simulink model "reduce_emf_before_speedloop"  (R2024b)
settings: Solver=FixedStepAuto  StartTime=0.0  StopTime=25  FixedStep=Tsim  RelTol=1e-4  EnableMultiTasking=on
InitFcn:
  | clc;
  | clear;
  | %% Parameters of the motor
  | Tsim = 1e-6;
  | Tpwm=1e-4;
  | Ts = 1e-4;
  | R = 1.8665;
  | Rs=1.8665;
  | Ls=8.96e-3;
  | Ld = 8.96e-3;
  | Lq = 8.96e-3;
  | L1=(Ld +Lq )/2;
  | L2=(Lq -Ld )/2;
  | flux = 0.21;
  | F=0.00008;
  | J=0.003;
  | Np=4;
  | fpwm = 10e3;
  | Vdc=311;
  | wn=100;
  | %% Controller limiter                                                           % Maximum torque (Nm)
  | I_max = 7.5;                                                    % Maximum current (A)
  | V_max = Vdc/sqrt(3);
  | 
  | 
  | %% 转速环电流环带宽
  | wspd=20;
  | wcur=500;
  | 
  | %% LESO
  | w0=10000;
  | beta1=2*w0-R/Ld;
  | beta2=w0*w0;
  | %% IF启动
  | Iq_if=7;
  | we_if_acc=300;
  | we_if_max=180;
  | we_switch=150;
model workspace (MAT data in the model file):
  new = 0
undefined symbols (not defined in the file or in its folder): DiscIntNeverNeededParam
libraries: spsDCVoltageSourceLib x1, spsGroundLib x1, spsPermanentMagnetSynchronousMachineLib x1, simulink x1, spsUniversalBridgeLib x1, spspowerguiLib x1
(part 1 of 2)
settings Model: SimulationMode=accelerator  Creator=Lenovo  LastModifiedBy=azx
settings SolverCC: AlgebraicLoopSolver=TrustRegion
settings DataIOCC: ReturnWorkspaceOutputs=off
settings OptimizationCC: ReuseModelBlockBuffer=off
settings DebuggingCC: UnconnectedInputMsg=warning  UnconnectedOutputMsg=warning  UnconnectedLineMsg=warning
settings ModelReferenceCC: EnableRefExpFcnMdlSchedulingChecks=on
settings RTWCC: GPUComputeCapability=3.5

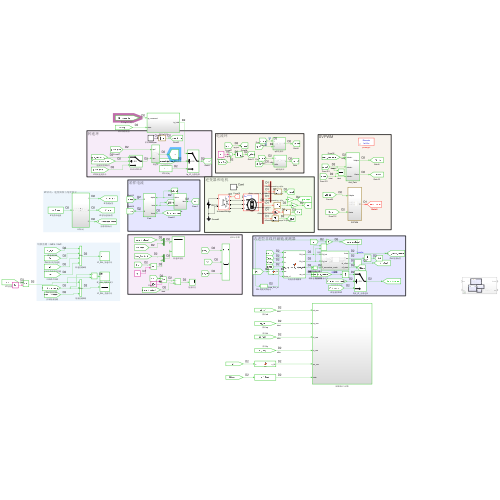
[thumbnail: Simulink's stored preview of the top-level diagram]
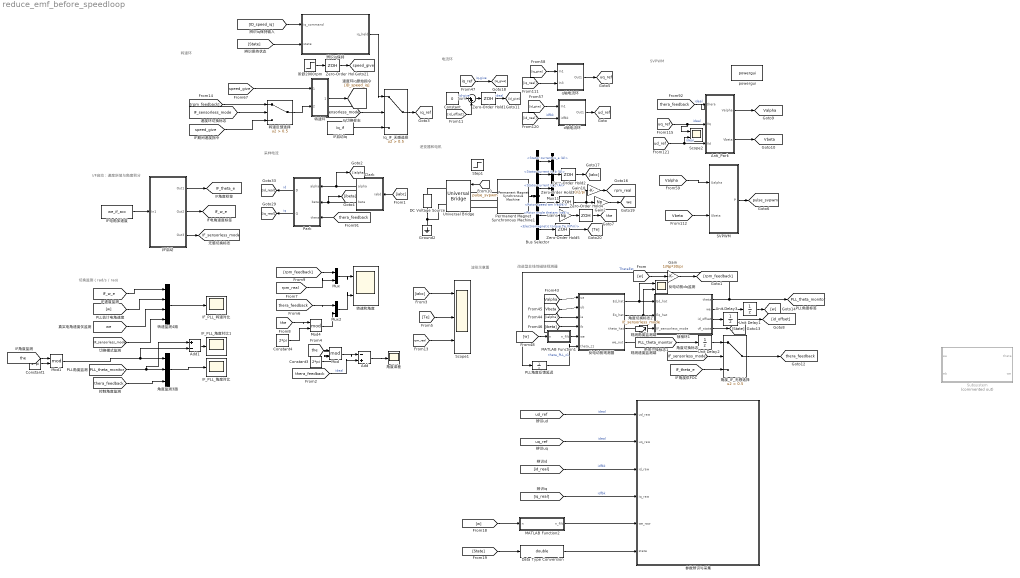
== system reduce_emf_before_speedloop ==
  note: 改进型非线性磁链观测器
  note: 波形示意图
  note: 采样电流
  note: 转速环
  note: SVPWM
  note: 逆变器和电机
  note: 电流环
  note: I/F启动：速度斜坡与角度积分
  note: 切换监测（rad/s / rad）
  Add : Sum  Inputs=-+
  Add1 : Sum  Inputs=+-
  Anti_Park : Subsystem
  Bus Selector : BusSelector  OutputSignals=Stator current is_a (A),Stator current is_b (A),Stator current is_c (A),Rotor speed wm (rad/s),Rotor angle thetam (rad),Electromagnetic torque Te (N*m)
  Clark : Subsystem
  Constant : Constant  Value=0
  Constant1 : Constant  Value=2*pi
  Constant3 : Constant  Value=2*pi
  Constant4 : Constant  Value=2*pi
  DC Voltage Source : spsDCVoltageSourceLib/DC Voltage Source  Amplitude=Vdc  Measurements=None
  Data Type Conversion : DataTypeConversion  OutDataTypeStr=double  SaturateOnIntegerOverflow=off  RndMeth=Floor
  Gain : Gain  Gain=1/Np*30/pi
  Gain10 : Gain  Gain=60/2/pi
  Gain2 : Gain  Gain=Np
  Gain5 : Gain  Gain=Np
  Ground2 : spsGroundLib/Ground  LConnTagsString=a
  I/F启动 : Subsystem
  IF_PLL_角度对比 : Scope
  IF_PLL_角度对比1 : Scope
  IF_PLL_转速对比 : Scope
  IF启动Iq : Constant  Value=Iq_if  SampleTime=Ts
  IF电角加速度 : Constant  Value=we_if_acc  SampleTime=Ts
  Iq_IF_无感选择 : Switch  Criteria=u2 > Threshold  Threshold=0.5
  MATLAB Function1 : MATLAB Function  Description=旁路100Hz低通，使用原有一拍延迟PLL速度，与角度反馈推进严格同拍。  TreatAsAtomicUnit=on
  MATLAB Function2 : MATLAB Function  TreatAsAtomicUnit=on
  Mod : Math  Operator=mod
  Mod1 : Math  Operator=mod
  Mod4 : Math  Operator=mod
  Mux : Mux  Inputs=2
  Mux11 : Mux  Inputs=3
  Mux2 : Mux  Inputs=2
  PLL角度反馈延迟 : UnitDelay  SampleTime=1e-4
  Park : Subsystem
  Permanent Magnet Synchronous Machine1 : spsPermanentMagnetSynchronousMachineLib/Permanent Magnet Synchronous Machine  NbPhases=3  FluxDistribution=Sinusoidal  RotorType=Salient-pole  MechanicalLoad=Torque Tm  PresetModel=No  ShowDetailedParameters=on  MeasurementBus=off  Resistance=R  Inductance=8.5e-3  dqInductances=[Ld,Lq]  La=Ld  MachineConstant=Flux linkage established by magnets (V.s)  Flux=0.21  VoltageCst=152.3591  TorqueCst=1.26  Flat=120  Mechanical=[0.03 2e-2 Np 0]  PolePairs=4  InitialConditions=[0,0, 0,0]  InitialConditions5ph=[0 0 0 0 0 0]  RefAngle=Aligned with phase A axis (original Park)  IterativeDiscreteModel=Trapezoidal non iterative  TsBlock=-1  TsPowergui=0
  SVPWM : Subsystem
  Scope1 : Scope  NumInputPorts=3
  Scope2 : Scope  NumInputPorts=2
  Step1 : Step  Time=0.5  Before=8.5  After=8.5  SampleTime=0
  Subsystem : Subsystem  Commented=on
  Sum : Sum  Inputs=|++
  Unit Delay1 : UnitDelay  SampleTime=-1  HasFrameUpgradeWarning=on
  Unit Delay2 : UnitDelay  SampleTime=-1  HasFrameUpgradeWarning=on
  Unit Delay3 : UnitDelay  SampleTime=-1  HasFrameUpgradeWarning=on
  Universal Bridge : spsUniversalBridgeLib/Universal Bridge  Arms=3  SnubberResistance=1e5  SnubberCapacitance=inf  Device=IGBT / Diodes  Ron=1e-3  Lon=0  ForwardVoltages="[  0  0  ]"  ForwardVoltage=0  GTOparameters=[ 10e-6 , 20e-6 ]  IGBTparameters=[ 1e-6 , 2e-6 ]  Measurements=None  Measurements_2=None  converterType=Rectifier
  Zero-Order Hold{,1..5} (6 alike) : ZeroOrderHold  SampleTime=1e-4
  d轴电流环 : Subsystem
  powergui : spspowerguiLib/powergui  Priority=1  SimulationMode=Discrete  SampleTime=Tsim  frequency=60  Iterations=50  frequencyindice=0  Pbase=100e6  ErrMax=1e-4  UnitsV=kV  UnitsW=MW  buscounter=0  FunctionMessages=off  echomessages=off  EnableUseOfTLC=off  CurrentSourceSwitches=off  DisableSnubberDevices=off  DisableRonSwitches=off  DisableVfSwitches=off  DisplayEquations=off  AutomaticDiscreteSolvers=off  SolverType=Tustin/Backward Euler (TBE)  Interpol=off  ExternalGateDelay=off  methode=off  Ts=100  x0status=blocks  SPID=on  SwTol=0  HookPort=off  NonlinearTolerance=1e-4  nMaxIteration=100  ContinueOnMaxIteration=off  RestoreLinks=warning  ResistiveCurrentMeasurement=off  Frange=[0:2:500]  Ylog=off  Xlog=on  ShowGrid=off  save=off  variable=ZData  structure=0  ZoomFFT=off  StartTime=0.0  cycles=1  DisplayStyle=1  fundamental=60  FreqAxis=off  MaxFrequency=1000  frequencyindicesteady=1  RmsSteady=1  display=off
  q轴电流环 : Subsystem
  参数辨识与采集 : Subsystem
  反电动势dq监测 : Scope  NumInputPorts=2
  反电动势观测器 : MATLAB Function  Description=按文档式12.5-12.7、图12.2实现dq降阶反电动势观测器，Ed/Eq直接送PLL。  TreatAsAtomicUnit=on
  观测角度监测端 : Terminator
  观测速度监测端 : Terminator
  角度_IF_无感选择 : Switch  Criteria=u2 > Threshold  Threshold=0.5
  角度监测3路 : Mux  Inputs=3
  角度误差 : Scope
  转速反馈选择 : Switch  Criteria=u2 > Threshold  Threshold=0.5
  转速和角度 : Scope  NumInputPorts=2
  转速环 : Subsystem
  转速监测4路 : Mux
  辨识iq保持 : Subsystem
  锁相环1 : Subsystem  Description=v2: 每段0.7s，前0.5s稳定、后0.2s采集；2~4与6~8期间保持iq指令，状态9逐点递推。
  阶跃2000rpm : Step  Time=2  Before=500  After=500  SampleTime=0
  tag scope: IF_sensorless_mode=global, IF_theta_e=global, IF_w_e=global, PLL_theta_monitor=global, Valpha=global, Vbeta=global, iq_ref=global, pulse_svpwm=global, rpm_real=global, speed_give=global, the=global, thera_feedback=global, ud_ref=global, uq_ref=global, we=global
  wires:
  [pulse_svpwm] -> Universal Bridge/1
  Clark/2(beta) -> [ibeta], Park/2(beta)
  Clark/1(alpha) -> [ialpha], Park/1(alpha)
  Park/1(D) -> [id_real]  "id"
  Park/2(Q) -> [iq_real]  "iq"
  阶跃2000rpm/1 -> Zero-Order Hold/1
  [thera_feedback] -> Park/3(thera)
  [thera_feedback] -> Anti_Park/1(thera)  "ideal"
  [ud_ref] -> Scope2/2, Anti_Park/3(Vd)  "ideal"
  [uq_ref] -> Scope2/1, Anti_Park/2(Vq)  "ideal"
  [iabc] -> Clark/1(iabd)
  Zero-Order Hold/1 -> [speed_give]
  Zero-Order Hold1/1 -> [id_give]  "ideal"
  Bus Selector/1 -> Mux11/1  "<Stator current is_a (A)>"
  Bus Selector/3 -> Mux11/3  "<Stator current is_c (A)>"
  Zero-Order Hold3/1 -> Gain2/1, Gain10/1
  Zero-Order Hold5/1 -> [Te]
  Gain2/1 -> [we]
  Mux11/1 -> Zero-Order Hold2/1
  Bus Selector/2 -> Mux11/2  "<Stator current is_b (A)>"
  Bus Selector/5 -> Gain5/1  "<Rotor angle thetam (rad)>"
  Bus Selector/4 -> Zero-Order Hold3/1  "<Rotor speed wm (rad/s)>"
  Bus Selector/6 -> Zero-Order Hold5/1  "<Electromagnetic torque Te (N*m)>"
  Zero-Order Hold2/1 -> [iabc]
  Gain10/1 -> [rpm_real]
  Permanent Magnet Synchronous Machine1/1 -> Bus Selector/1
  Zero-Order Hold4/1 -> [the]
  Gain5/1 -> Zero-Order Hold4/1
  [rpm_feedback] -> Mux/1
  [rpm_real] -> Mux/2
  [thera_feedback] -> Mux2/1
  Mux2/1 -> 转速和角度/2
  Mux/1 -> 转速和角度/1
  [the] -> Mod/1
  Constant3/1 -> Mod/2
  Mod/1 -> Add/1
  Add/1 -> 角度误差/1
  Anti_Park/1(Valpha) -> [Valpha]
  Anti_Park/2(Vbeta) -> [Vbeta]
  [thera_feedback] -> Add/2  "ideal"
  [the] -> Mod4/1
  Constant4/1 -> Mod4/2
  Mod4/1 -> Mux2/2
  [speed_give] -> 转速环/1(rpm*)
  [iq_give] -> q轴电流环/1(In1)
  [iq_real] -> q轴电流环/2(In3)
  q轴电流环/1(Out1) -> [uq_ref]
  [id_give] -> d轴电流环/1(In1)
  [id_real] -> d轴电流环/2(idfbk)  "idfbk"
  d轴电流环/1(Out1) -> [ud_ref]
  SVPWM/1(P) -> [pulse_svpwm]
  [rpm_real] -> Scope1/3
  [Te] -> Scope1/2
  [iabc] -> Scope1/1
  Gain/1 -> [rpm_feedback]
  [Valpha] -> 反电动势观测器/1(ua)
  反电动势观测器/2(Eq_hat) -> 锁相环1/2(Eq_hat), 反电动势dq监测/2
  [Vbeta] -> 反电动势观测器/2(ub)
  [ialpha] -> 反电动势观测器/3(ia)
  [ibeta] -> 反电动势观测器/4(ib)
  反电动势观测器/1(Ed_hat) -> 锁相环1/1(Ed_hat), 反电动势dq监测/1
  Unit Delay1/1 -> [w]
  角度_IF_无感选择/1 -> [thera_feedback]
  [Valpha] -> SVPWM/1(Ualpha)
  [Vbeta] -> SVPWM/2(Ubeta)
  锁相环1/2(we) -> Unit Delay1/1
  [w] -> MATLAB Function1/1(n)
  [w] -> Gain/1
  [IF_sensorless_mode] -> Iq_IF_无感选择/2
  IF启动Iq/1 -> Iq_IF_无感选择/3
  Iq_IF_无感选择/1 -> [iq_ref]
  [rpm_feedback] -> 转速反馈选择/1
  [IF_sensorless_mode] -> 转速反馈选择/2
  [speed_give] -> 转速反馈选择/3
  转速反馈选择/1 -> 转速环/2(rpm)
  锁相环1/1(theta) -> [PLL_theta_monitor], PLL角度反馈延迟/1  "ThetaEst"
  [IF_sensorless_mode] -> 角度_IF_无感选择/2
  [IF_theta_e] -> 角度_IF_无感选择/3
  [IF_w_e] -> 转速监测4路/1
  [w] -> 转速监测4路/2
  [we] -> 转速监测4路/3
  [IF_sensorless_mode] -> 转速监测4路/4
  转速监测4路/1 -> IF_PLL_转速对比/1
  [PLL_theta_monitor] -> Add1/1, 角度监测3路/2
  [thera_feedback] -> 角度监测3路/3
  角度监测3路/1 -> IF_PLL_角度对比/1
  [PLL_theta_monitor] -> Unit Delay2/1
  IF电角加速度/1 -> I/F启动/1(In1)
  I/F启动/1(Out1) -> [IF_theta_e]
  I/F启动/2(Out2) -> [IF_w_e]
  I/F启动/3(Out3) -> [IF_sensorless_mode]
  [IF_sensorless_mode] -> 锁相环1/3(IF_sensorless_mode)
  锁相环1/3(id_offset) -> Unit Delay3/1
  Sum/1 -> Zero-Order Hold1/1
  Constant/1 -> Sum/1  "id-give"
  [id_offset] -> Sum/2
  Unit Delay3/1 -> [id_offset]
  [w] -> MATLAB Function2/1(n)
  锁相环1/4(vfl_state) -> [State]
  [State] -> Data Type Conversion/1
  Add1/1 -> IF_PLL_角度对比1/1
  [the] -> Mod1/1
  Constant1/1 -> Mod1/2
  Mod1/1 -> Add1/2, 角度监测3路/1
  MATLAB Function1/1(n_filt) -> 反电动势观测器/5("we ")
  Unit Delay2/1 -> 角度_IF_无感选择/1
  PLL角度反馈延迟/1 -> 反电动势观测器/6(theta_z1)  "theta_PLL_z1"
  反电动势观测器/3(theta_hat) -> 观测角度监测端/1
  反电动势观测器/4(we_out) -> 观测速度监测端/1
  [ud_ref] -> 参数辨识与采集/1(ud_raw)  "ideal"
  [uq_ref] -> 参数辨识与采集/2(uq_raw)  "ideal"
  [id_real] -> 参数辨识与采集/3(id_raw)  "idfbk"
  [iq_real] -> 参数辨识与采集/4(iq_raw)  "idfbk"
  MATLAB Function2/1(n_filt) -> 参数辨识与采集/5(we_raw)
  Data Type Conversion/1 -> 参数辨识与采集/6(state)
  [State] -> 辨识iq保持/2(state)
  辨识iq保持/1(iq_held) -> Iq_IF_无感选择/1
  [iq_ref] -> [iq_give]  "iq-give"
  转速环/1(Out1) -> [ID_speed_iq]
  [ID_speed_iq] -> 辨识iq保持/1(iq_command)
  connections:
  DC Voltage Source/RConn1 -- Universal Bridge/RConn1
  Permanent Magnet Synchronous Machine1/LConn1 -- Universal Bridge/LConn1
  Permanent Magnet Synchronous Machine1/LConn2 -- Universal Bridge/LConn2
  Permanent Magnet Synchronous Machine1/LConn3 -- Universal Bridge/LConn3
  Universal Bridge/RConn2 -- DC Voltage Source/LConn1 -- Ground2/LConn1

== system reduce_emf_before_speedloop/Anti_Park ==
  thera : Inport
  Vq : Inport  Port=2
  Vd : Inport  Port=3
  Fcn : Fcn  Expr=cos(u[1])*u[2]-sin(u[1])*u[3]
  Fcn1 : Fcn  Expr=sin(u[1])*u[2]+cos(u[1])*u[3]
  Mux1 : Mux  Inputs=3
  Valpha : Outport
  Vbeta : Outport  Port=2
  wires:
  thera/1 -> Mux1/1
  Mux1/1 -> Fcn1/1, Fcn/1
  Vq/1 -> Mux1/3
  Fcn1/1 -> Vbeta/1
  Vd/1 -> Mux1/2
  Fcn/1 -> Valpha/1

== system reduce_emf_before_speedloop/Clark ==
  iabd : Inport
  Fcn : Fcn  Expr=(u(1)-0.5*(u(2)+u(3)))*2/3
  Fcn1 : Fcn  Expr=sqrt(3)/2*(u(2)-u(3))*2/3
  alpha : Outport
  beta : Outport  Port=2
  tag scope: Ialpha_real=global, Ibeta_real=global
  wires:
  iabd/1 -> Fcn1/1, Fcn/1
  Fcn/1 -> [Ialpha_real], alpha/1
  Fcn1/1 -> [Ibeta_real], beta/1

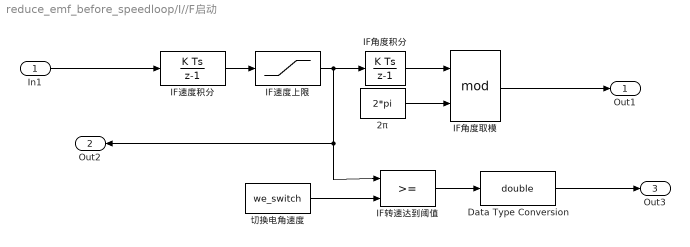
== system reduce_emf_before_speedloop/I//F启动 ==
  In1 : Inport
  2π : Constant  Value=2*pi  SampleTime=Ts
  Data Type Conversion : DataTypeConversion  OutDataTypeStr=double  SaturateOnIntegerOverflow=off  RndMeth=Floor
  IF角度取模 : Math  Operator=mod
  IF角度积分 : DiscreteIntegrator  SampleTime=Ts  ICPrevOutput=DiscIntNeverNeededParam  ICPrevScaledInput=DiscIntNeverNeededParam
  IF转速达到阈值 : RelationalOperator
  IF速度上限 : Saturate  UpperLimit=we_if_max  LowerLimit=0
  IF速度积分 : DiscreteIntegrator  SampleTime=Ts  ICPrevOutput=DiscIntNeverNeededParam  ICPrevScaledInput=DiscIntNeverNeededParam
  切换电角速度 : Constant  Value=we_switch  SampleTime=Ts
  Out1 : Outport
  Out2 : Outport  Port=2
  Out3 : Outport  Port=3
  wires:
  切换电角速度/1 -> IF转速达到阈值/2
  IF速度积分/1 -> IF速度上限/1
  2π/1 -> IF角度取模/2
  IF速度上限/1 -> Out2/1, IF转速达到阈值/1, IF角度积分/1
  IF角度积分/1 -> IF角度取模/1
  IF转速达到阈值/1 -> Data Type Conversion/1
  In1/1 -> IF速度积分/1
  Data Type Conversion/1 -> Out3/1
  IF角度取模/1 -> Out1/1

== system reduce_emf_before_speedloop/Park ==
  alpha : Inport
  beta : Inport  Port=2
  thera : Inport  Port=3
  Fcn : Fcn  Expr=u(1)*cos(u(3))+u(2)*sin(u(3))
  Fcn1 : Fcn  Expr=-u(1)*sin(u(3))+u(2)*cos(u(3))
  Mux1 : Mux  Inputs=3
  D : Outport
  Q : Outport  Port=2
  wires:
  beta/1 -> Mux1/2
  Mux1/1 -> Fcn1/1, Fcn/1
  thera/1 -> Mux1/3
  Fcn/1 -> D/1
  Fcn1/1 -> Q/1
  alpha/1 -> Mux1/1

== system reduce_emf_before_speedloop/SVPWM ==
  Ualpha : Inport
  Ubeta : Inport  Port=2
  Rate Transition : RateTransition  Deterministic=off
  Rate Transition12 : RateTransition  Deterministic=off
  SVPWM : Subsystem
  P : Outport
  wires:
  Ualpha/1 -> Rate Transition/1
  Ubeta/1 -> Rate Transition12/1
  Rate Transition/1 -> SVPWM/1(alpha)
  Rate Transition12/1 -> SVPWM/2(beta)
  SVPWM/1(Pulse) -> P/1

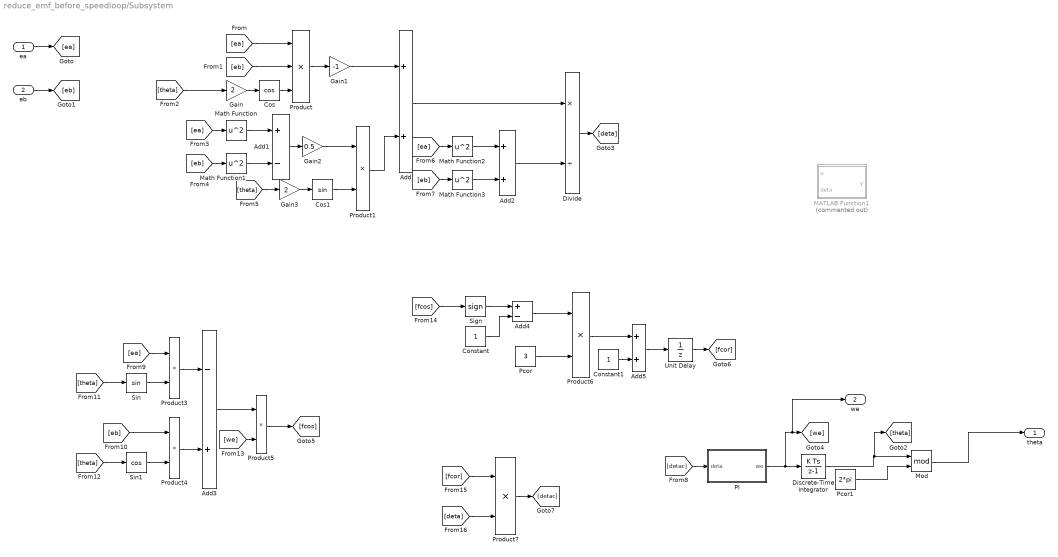
== system reduce_emf_before_speedloop/Subsystem ==
  ea : Inport
  eb : Inport  Port=2
  Add : Sum
  Add1 : Sum  Inputs=+-
  Add2 : Sum
  Add3 : Sum  Inputs=-+
  Add4 : Sum  Inputs=+-
  Add5 : Sum
  Constant : Constant
  Constant1 : Constant
  Cos : Trigonometry  Operator=cos
  Cos1 : Trigonometry
  Discrete-Time Integrator : DiscreteIntegrator  SampleTime=-1  ICPrevOutput=DiscIntNeverNeededParam  ICPrevScaledInput=DiscIntNeverNeededParam
  Divide : Product  Inputs=*/
  Gain : Gain  Gain=2
  Gain1 : Gain  Gain=-1
  Gain2 : Gain  Gain=0.5
  Gain3 : Gain  Gain=2
  MATLAB Function1 : MATLAB Function  Commented=on  TreatAsAtomicUnit=on
  Math Function{,1..3} (4 alike) : Math  Operator=square
  Mod : Math  Operator=mod
  PI : Subsystem
  Pcor : Constant  Value=3
  Pcor1 : Constant  Value=2*pi
  Product : Product  Inputs=3
  Product{1,3..7} (6 alike) : Product
  Sign : Signum
  Sin : Trigonometry
  Sin1 : Trigonometry  Operator=cos
  Unit Delay : UnitDelay  SampleTime=-1  HasFrameUpgradeWarning=on
  theta : Outport
  we : Outport  Port=2
  wires:
  ea/1 -> [ea]
  eb/1 -> [eb]
  [ea] -> Product/1
  [eb] -> Product/2
  Cos/1 -> Product/3
  Gain/1 -> Cos/1
  [theta] -> Gain/1
  Product/1 -> Gain1/1
  Gain1/1 -> Add/1
  [ea] -> Math Function/1
  [eb] -> Math Function1/1
  Math Function/1 -> Add1/1
  Math Function1/1 -> Add1/2
  Add1/1 -> Gain2/1
  Gain2/1 -> Product1/1
  Product1/1 -> Add/2
  Cos1/1 -> Product1/2
  Gain3/1 -> Cos1/1
  [theta] -> Gain3/1
  Add/1 -> Divide/1
  Math Function3/1 -> Add2/2
  [ea] -> Math Function2/1
  [eb] -> Math Function3/1
  Math Function2/1 -> Add2/1
  [ea] -> Product3/1
  Sin/1 -> Product3/2
  [theta] -> Sin/1
  [eb] -> Product4/1
  [theta] -> Sin1/1
  Sin1/1 -> Product4/2
  Product3/1 -> Add3/1
  Product4/1 -> Add3/2
  Add3/1 -> Product5/1
  [we] -> Product5/2
  Product5/1 -> [fcos]
  [fcos] -> Sign/1
  Sign/1 -> Add4/1
  Constant/1 -> Add4/2
  Add4/1 -> Product6/1
  Pcor/1 -> Product6/2
  Product6/1 -> Add5/1
  Constant1/1 -> Add5/2
  Add5/1 -> Unit Delay/1
  [fcor] -> Product7/1
  [deta] -> Product7/2
  Product7/1 -> [detac]
  PI/1(we) -> Discrete-Time Integrator/1, we/1, [we]
  Discrete-Time Integrator/1 -> [theta], Mod/1
  Unit Delay/1 -> [fcor]
  Pcor1/1 -> Mod/2
  [detac] -> PI/1(deta)
  Add2/1 -> Divide/2
  Divide/1 -> [deta]
  Mod/1 -> theta/1

== system reduce_emf_before_speedloop/d轴电流环 ==
  In1 : Inport
  idfbk : Inport  Port=2
  30id : Subsystem  DialogController=POWERSYS.PowerSysDialog  mask(Discrete PI Controller){Kp=2*pi*wcur*Ld, Ki=2*pi*wcur*R, Par_Limits=[V_max -V_max], Init=0, Ts=Ts}
      mask prompts: Kp "Proportional gain (Kp):"; Ki "Integral gain (Ki):"; Par_Limits "Output limits: [ Upper   Lower ]"; Init "Output initial value:"; Ts "Sample time:"
      mask help: This block implements a discrete PI controller.
      mask init:
      | UpperLimit=Par_Limits(1);
      | LowerLimit=Par_Limits(2);
      | power_initmask();
      mask Help: This block is part of a subset of blocks in the Extras library that does not have documentation associated with it, other than the block mask description.
      mask Display: disp('PI');
  Sum1 : Sum  Inputs=|+-
  Sum7 : Sum  Inputs=|+-
  Out1 : Outport
  wires:
  30id/1(Out) -> Sum7/1  "ideal"
  Sum1/1 -> 30id/1(Error)
  Sum7/1 -> Out1/1
  idfbk/1 -> Sum1/2
  In1/1 -> Sum1/1

== system reduce_emf_before_speedloop/q轴电流环 ==
  In1 : Inport
  In3 : Inport  Port=2
  30iq : Subsystem  DialogController=POWERSYS.PowerSysDialog  mask(Discrete PI Controller){Kp=2*pi*wcur*Lq, Ki=2*pi*wcur*R, Par_Limits=[V_max -V_max], Init=0, Ts=Ts}
      mask prompts: Kp "Proportional gain (Kp):"; Ki "Integral gain (Ki):"; Par_Limits "Output limits: [ Upper   Lower ]"; Init "Output initial value:"; Ts "Sample time:"
      mask help: This block implements a discrete PI controller.
      mask init:
      | UpperLimit=Par_Limits(1);
      | LowerLimit=Par_Limits(2);
      | power_initmask();
      mask Help: This block is part of a subset of blocks in the Extras library that does not have documentation associated with it, other than the block mask description.
      mask Display: disp('PI');
  Sum2 : Sum  Inputs=|+-
  Sum6 : Sum  Inputs=|++
  Out1 : Outport
  wires:
  In3/1 -> Sum2/2
  30iq/1(Out) -> Sum6/1  "ideal"
  Sum2/1 -> 30iq/1(Error)
  In1/1 -> Sum2/1
  Sum6/1 -> Out1/1

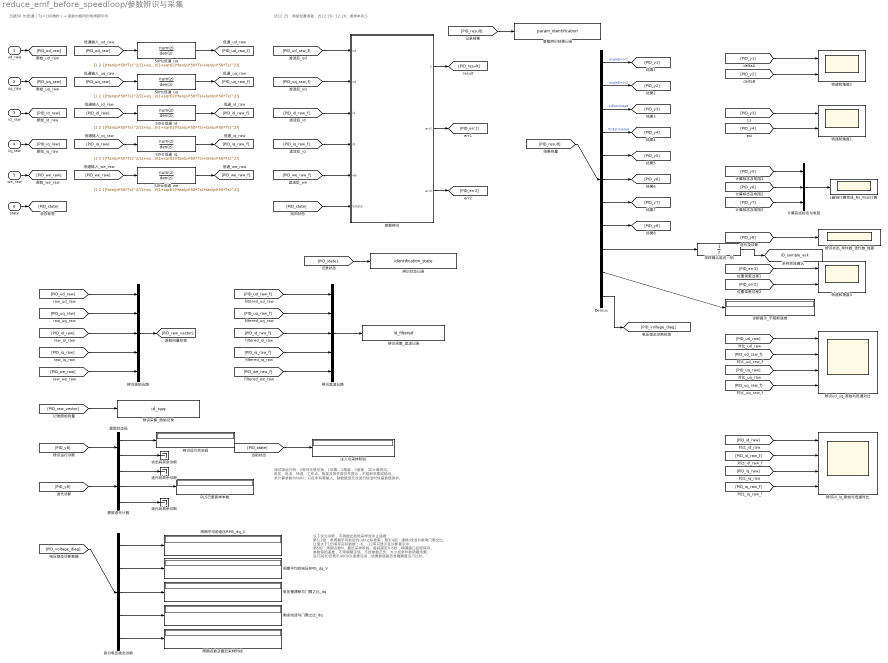
== system reduce_emf_before_speedloop/参数辨识与采集 ==
  note: 五路50 Hz低通（Ts=100微秒）→ 函数内相同的电周期平均
  note: 式12.25：两组位置误差；式12.26～12.28：逐样本RLS
  note: 调试版运行码：0等待无感切换，1采集，2角度，3递推，30计算完成。
      | 电压、电流、转速、工作点、角度及条件数仅作提示，不阻断采集或输出。
      | 未计算参数为NaN；只在非有限输入、缺数据或无法进行除法时保留数值保护。
  note: 以下仅为诊断，不再据此拒绝采样或中止递推：
      | 第1/2组：电周期平均前后的ud/uq标准差；第3/4组：漂移/纹波与参考门限之比。
      | 比值大于1仍保存实际数据；-6、-12等只显示在诊断提示中。
      | 第5组：周期点数N、最近采样阶段。每段固定0.6秒，填满窗口后即保存。
      | 参数每拍递推，不预填额定值，不按参数正负、大小或条件数隐藏结果。
      | 运行码30仅表示4000次递推完成，结果数值是否准确需要另行比对。
  ud_raw : Inport
  uq_raw : Inport  Port=2
  id_raw : Inport  Port=3
  iq_raw : Inport  Port=4
  we_raw : Inport  Port=5
  state : Inport  Port=6
  50Hz低通_id : DiscreteTransferFcn  Description=输入已是Ts=100us；同速率二阶Butterworth低通，不作升采样，不声称恢复上游已混叠信息。  Numerator=[1 2 1]*tan(pi*50*Ts)^2/(1+sqrt(2)*tan(pi*50*Ts)+tan(pi*50*Ts)^2)  Denominator=[1 2*(tan(pi*50*Ts)^2-1)/(1+sqrt(2)*tan(pi*50*Ts)+tan(pi*50*Ts)^2) (1-sqrt(2)*tan(pi*50*Ts)+tan(pi*50*Ts)^2)/(1+sqrt(2)*tan(pi*50*Ts)+tan(pi*50*Ts)^2)]  SampleTime=Ts
  50Hz低通_iq : DiscreteTransferFcn  Description=输入已是Ts=100us；同速率二阶Butterworth低通，不作升采样，不声称恢复上游已混叠信息。  Numerator=[1 2 1]*tan(pi*50*Ts)^2/(1+sqrt(2)*tan(pi*50*Ts)+tan(pi*50*Ts)^2)  Denominator=[1 2*(tan(pi*50*Ts)^2-1)/(1+sqrt(2)*tan(pi*50*Ts)+tan(pi*50*Ts)^2) (1-sqrt(2)*tan(pi*50*Ts)+tan(pi*50*Ts)^2)/(1+sqrt(2)*tan(pi*50*Ts)+tan(pi*50*Ts)^2)]  SampleTime=Ts
  50Hz低通_ud : DiscreteTransferFcn  Description=输入已是Ts=100us；同速率二阶Butterworth低通，不作升采样，不声称恢复上游已混叠信息。  Numerator=[1 2 1]*tan(pi*50*Ts)^2/(1+sqrt(2)*tan(pi*50*Ts)+tan(pi*50*Ts)^2)  Denominator=[1 2*(tan(pi*50*Ts)^2-1)/(1+sqrt(2)*tan(pi*50*Ts)+tan(pi*50*Ts)^2) (1-sqrt(2)*tan(pi*50*Ts)+tan(pi*50*Ts)^2)/(1+sqrt(2)*tan(pi*50*Ts)+tan(pi*50*Ts)^2)]  SampleTime=Ts
  50Hz低通_uq : DiscreteTransferFcn  Description=输入已是Ts=100us；同速率二阶Butterworth低通，不作升采样，不声称恢复上游已混叠信息。  Numerator=[1 2 1]*tan(pi*50*Ts)^2/(1+sqrt(2)*tan(pi*50*Ts)+tan(pi*50*Ts)^2)  Denominator=[1 2*(tan(pi*50*Ts)^2-1)/(1+sqrt(2)*tan(pi*50*Ts)+tan(pi*50*Ts)^2) (1-sqrt(2)*tan(pi*50*Ts)+tan(pi*50*Ts)^2)/(1+sqrt(2)*tan(pi*50*Ts)+tan(pi*50*Ts)^2)]  SampleTime=Ts
  50Hz低通_we : DiscreteTransferFcn  Description=输入已是Ts=100us；同速率二阶Butterworth低通，不作升采样，不声称恢复上游已混叠信息。  Numerator=[1 2 1]*tan(pi*50*Ts)^2/(1+sqrt(2)*tan(pi*50*Ts)+tan(pi*50*Ts)^2)  Denominator=[1 2*(tan(pi*50*Ts)^2-1)/(1+sqrt(2)*tan(pi*50*Ts)+tan(pi*50*Ts)^2) (1-sqrt(2)*tan(pi*50*Ts)+tan(pi*50*Ts)^2)/(1+sqrt(2)*tan(pi*50*Ts)+tan(pi*50*Ts)^2)]  SampleTime=Ts
  Demux : Demux  Outputs=[1 1 1 1 1 1 1 8 1 1 10]
  L磁链计算完成_Rs_Rs已计算 : Scope
  RLS已更新样本数 : Display
  剩余纹波与门限之比_dq : Display
  参数辨识 : MATLAB Function  Description=v7调试版：填满窗口即保存，质量诊断不拒绝数据；按真实存储数据执行4000次递推。运行码30表示递推完成，计算标志不表示通过精度或物理验收。  TreatAsAtomicUnit=on
  参数辨识结果记录 : ToWorkspace  VariableName=param_identification  SaveFormat=Structure With Time  SampleTime=Ts
  周期平均前电压RMS_dq_V : Display
  周期平均后电压RMS_dq_V : Display
  周期点数及最近采样阶段 : Display
  拆分电压稳态诊断 : Demux  Outputs=[2 2 2 2 2]
  提取状态码 : Demux  Outputs=[1 7]
  提取迭代计数 : Demux  Outputs=[4 1 3]
  注入与采样阶段 : Display
  状态码其余诊断 : Terminator
  电压慢漂移与门限之比_dq : Display
  计算完成标志与电阻 : Mux  Inputs=3
  诊断提示_不阻断递推 : Display
  转速和角度1 : Scope  NumInputPorts=2
  转速和角度2 : Scope  NumInputPorts=2
  转速和角度4 : Scope  NumInputPorts=2
  辨识id_iq_原始与低通对比 : Scope
  辨识ud_uq_原始与低通对比 : Scope
  辨识原始五路 : Mux  Inputs=5
  辨识滤波五路 : Mux  Inputs=5
  辨识状态_条件数_迭代数_残差 : Scope
  辨识状态记录 : ToWorkspace  VariableName=identification_state  SaveFormat=Structure With Time  SampleTime=Ts
  辨识运行状态码 : Display
  辨识采集_原始记录 : ToWorkspace  VariableName=id_raw  SaveFormat=Structure With Time  SampleTime=Ts
  辨识采集_滤波记录 : ToWorkspace  VariableName=id_filtered  SaveFormat=Structure With Time  SampleTime=Ts
  迭代前其余诊断 : Terminator
  迭代后其余诊断 : Terminator
  采样确认延迟一拍 : UnitDelay  SampleTime=Ts
  tag scope: ID_sample_ack=global
  wires:
  参数辨识/1(y) -> [PID_result]
  参数辨识/2(err1) -> [PID_err1]
  参数辨识/3(err2) -> [PID_err2]
  [PID_result] -> Demux/1
  Demux/1 -> [PID_y1]  "angleError1"
  Demux/2 -> [PID_y2]  "angleError2"
  Demux/3 -> [PID_y3]  "LsEstimated"
  Demux/4 -> [PID_y4]  "PsiEstimated"
  Demux/5 -> [PID_y5]
  Demux/6 -> [PID_y6]
  Demux/7 -> [PID_y7]
  Demux/8 -> [PID_y8]
  [PID_result] -> 参数辨识结果记录/1
  [PID_state] -> 辨识状态记录/1
  [PID_y1] -> 转速和角度2/1
  [PID_y2] -> 转速和角度2/2
  [PID_y3] -> 转速和角度1/1
  [PID_y4] -> 转速和角度1/2
  [PID_y5] -> 计算完成标志与电阻/1
  [PID_y6] -> 计算完成标志与电阻/2
  [PID_y7] -> 计算完成标志与电阻/3
  计算完成标志与电阻/1 -> L磁链计算完成_Rs_Rs已计算/1
  [PID_y8] -> 辨识状态_条件数_迭代数_残差/1
  [PID_err1] -> 转速和角度4/1
  [PID_err2] -> 转速和角度4/2
  [PID_ud_raw] -> 辨识原始五路/1
  [PID_uq_raw] -> 辨识原始五路/2
  [PID_id_raw] -> 辨识原始五路/3
  [PID_iq_raw] -> 辨识原始五路/4
  [PID_we_raw] -> 辨识原始五路/5
  辨识滤波五路/1 -> 辨识采集_滤波记录/1
  [PID_ud_raw_f] -> 辨识滤波五路/1
  [PID_uq_raw_f] -> 辨识滤波五路/2
  [PID_id_raw_f] -> 辨识滤波五路/3
  [PID_iq_raw_f] -> 辨识滤波五路/4
  [PID_we_raw_f] -> 辨识滤波五路/5
  [PID_ud_raw] -> 辨识ud_uq_原始与低通对比/1
  [PID_ud_raw_f] -> 辨识ud_uq_原始与低通对比/2
  [PID_uq_raw] -> 辨识ud_uq_原始与低通对比/3
  [PID_uq_raw_f] -> 辨识ud_uq_原始与低通对比/4
  [PID_id_raw] -> 辨识id_iq_原始与低通对比/1
  [PID_id_raw_f] -> 辨识id_iq_原始与低通对比/2
  [PID_iq_raw] -> 辨识id_iq_原始与低通对比/3
  [PID_iq_raw_f] -> 辨识id_iq_原始与低通对比/4
  辨识原始五路/1 -> [PID_raw_vector]
  [PID_raw_vector] -> 辨识采集_原始记录/1
  Demux/9 -> 采样确认延迟一拍/1
  采样确认延迟一拍/1 -> [ID_sample_ack]
  Demux/10 -> 诊断提示_不阻断递推/1
  [PID_state] -> 注入与采样阶段/1
  [PID_y8] -> 提取状态码/1
  提取状态码/1 -> 辨识运行状态码/1
  提取状态码/2 -> 状态码其余诊断/1
  [PID_y8] -> 提取迭代计数/1
  提取迭代计数/1 -> 迭代前其余诊断/1
  提取迭代计数/2 -> RLS已更新样本数/1
  提取迭代计数/3 -> 迭代后其余诊断/1
  ud_raw/1 -> [PID_ud_raw]
  [PID_ud_raw] -> 50Hz低通_ud/1
  50Hz低通_ud/1 -> [PID_ud_raw_f]
  [PID_ud_raw_f] -> 参数辨识/1(ud)
  uq_raw/1 -> [PID_uq_raw]
  [PID_uq_raw] -> 50Hz低通_uq/1
  50Hz低通_uq/1 -> [PID_uq_raw_f]
  [PID_uq_raw_f] -> 参数辨识/2(uq)
  id_raw/1 -> [PID_id_raw]
  [PID_id_raw] -> 50Hz低通_id/1
  50Hz低通_id/1 -> [PID_id_raw_f]
  [PID_id_raw_f] -> 参数辨识/3(id)
  iq_raw/1 -> [PID_iq_raw]
  [PID_iq_raw] -> 50Hz低通_iq/1
  50Hz低通_iq/1 -> [PID_iq_raw_f]
  [PID_iq_raw_f] -> 参数辨识/4(iq)
  we_raw/1 -> [PID_we_raw]
  [PID_we_raw] -> 50Hz低通_we/1
  50Hz低通_we/1 -> [PID_we_raw_f]
  [PID_we_raw_f] -> 参数辨识/5(we)
  state/1 -> [PID_state]
  [PID_state] -> 参数辨识/6(Vstate)
  Demux/11 -> [PID_voltage_diag]
  [PID_voltage_diag] -> 拆分电压稳态诊断/1
  拆分电压稳态诊断/1 -> 周期平均前电压RMS_dq_V/1
  拆分电压稳态诊断/2 -> 周期平均后电压RMS_dq_V/1
  拆分电压稳态诊断/3 -> 电压慢漂移与门限之比_dq/1
  拆分电压稳态诊断/4 -> 剩余纹波与门限之比_dq/1
  拆分电压稳态诊断/5 -> 周期点数及最近采样阶段/1

== system reduce_emf_before_speedloop/转速环 ==
  rpm* : Inport
  rpm : Inport  Port=2
  30speed : Subsystem  DialogController=POWERSYS.PowerSysDialog  mask(Discrete PI Controller){Kp=0.5, Ki=5, Par_Limits=[I_max -I_max], Init=0, Ts=Ts}
      mask prompts: Kp "Proportional gain (Kp):"; Ki "Integral gain (Ki):"; Par_Limits "Output limits: [ Upper   Lower ]"; Init "Output initial value:"; Ts "Sample time:"
      mask help: This block implements a discrete PI controller.
      mask init:
      | UpperLimit=Par_Limits(1);
      | LowerLimit=Par_Limits(2);
      | power_initmask();
      mask Help: This block is part of a subset of blocks in the Extras library that does not have documentation associated with it, other than the block mask description.
      mask Display: disp('PI');
  Gain : Gain  Gain=2*pi/60
  Sum : Sum  Inputs=|+-
  辨识期间暂停速度PI误差 : Switch  Criteria=u2 > Threshold  Threshold=0.5
  辨识期间零速度误差 : Constant  Value=0  SampleTime=Ts
  Out1 : Outport
  wires:
  Sum/1 -> Gain/1
  rpm*/1 -> Sum/1
  rpm/1 -> Sum/2
  Gain/1 -> 辨识期间暂停速度PI误差/3
  30speed/1(Out) -> Out1/1
  [ID_acquisition_hold] -> 辨识期间暂停速度PI误差/2
  辨识期间零速度误差/1 -> 辨识期间暂停速度PI误差/1
  辨识期间暂停速度PI误差/1 -> 30speed/1(Error)

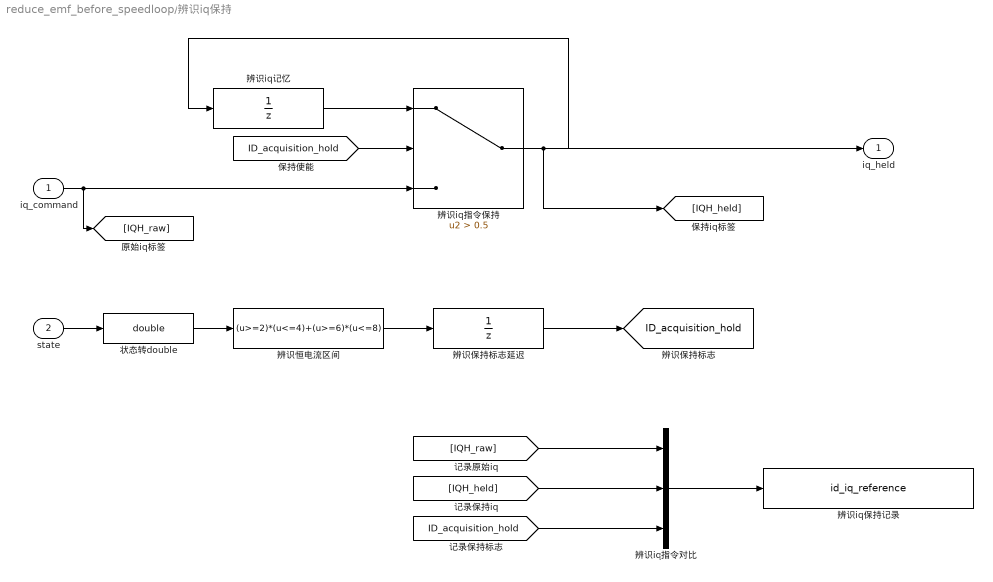
== system reduce_emf_before_speedloop/辨识iq保持 ==
  iq_command : Inport
  state : Inport  Port=2
  状态转double : DataTypeConversion  OutDataTypeStr=double
  辨识iq保持记录 : ToWorkspace  VariableName=id_iq_reference  SaveFormat=Structure With Time  SampleTime=Ts
  辨识iq指令保持 : Switch  Criteria=u2 > Threshold  Threshold=0.5
  辨识iq指令对比 : Mux  Inputs=3
  辨识iq记忆 : UnitDelay  SampleTime=Ts
  辨识保持标志延迟 : UnitDelay  SampleTime=Ts
  辨识恒电流区间 : Fcn  Expr=(u>=2)*(u<=4)+(u>=6)*(u<=8)
  iq_held : Outport
  tag scope: ID_acquisition_hold=global
  wires:
  state/1 -> 状态转double/1
  状态转double/1 -> 辨识恒电流区间/1
  iq_command/1 -> 辨识iq指令保持/3, [IQH_raw]
  辨识恒电流区间/1 -> 辨识保持标志延迟/1
  辨识保持标志延迟/1 -> [ID_acquisition_hold]
  [ID_acquisition_hold] -> 辨识iq指令保持/2
  辨识iq记忆/1 -> 辨识iq指令保持/1
  辨识iq指令保持/1 -> 辨识iq记忆/1, iq_held/1, [IQH_held]
  [IQH_raw] -> 辨识iq指令对比/1
  [IQH_held] -> 辨识iq指令对比/2
  [ID_acquisition_hold] -> 辨识iq指令对比/3
  辨识iq指令对比/1 -> 辨识iq保持记录/1

== system reduce_emf_before_speedloop/锁相环1 ==
  Ed_hat : Inport
  Eq_hat : Inport  Port=2
  IF_sensorless_mode : Inport  Port=3
  MATLAB Function : MATLAB Function  TreatAsAtomicUnit=on
  theta : Outport
  we : Outport  Port=2
  id_offset : Outport  Port=3
  vfl_state : Outport  Port=4
  wires:
  Ed_hat/1 -> MATLAB Function/1(Ed_hat)
  Eq_hat/1 -> MATLAB Function/2(Eq_hat)
  MATLAB Function/1(theta) -> theta/1
  MATLAB Function/2(we) -> we/1
  IF_sensorless_mode/1 -> MATLAB Function/3(IF_sensorless_mode)
  MATLAB Function/3(id_offset) -> id_offset/1
  MATLAB Function/4(vfl_state) -> vfl_state/1
  [ID_sample_ack] -> MATLAB Function/4(sample_ack)

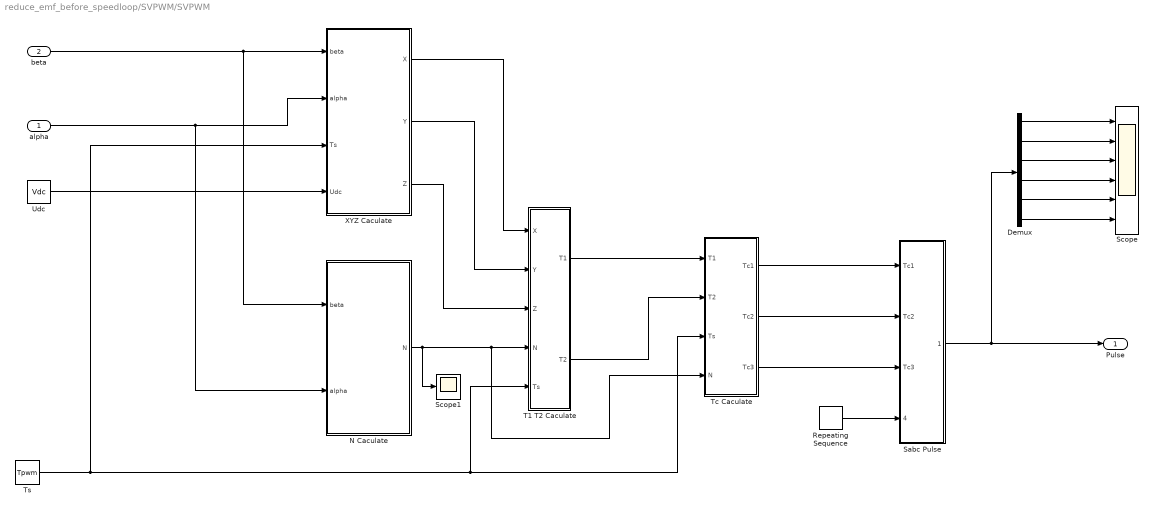
== system reduce_emf_before_speedloop/SVPWM/SVPWM ==
  alpha : Inport
  beta : Inport  Port=2
  Demux : Demux  Outputs=6
  N Caculate : Subsystem
  Repeating Sequence : simulink/Sources/Repeating Sequence  rep_seq_t=[0 0.5*Tpwm Tpwm]  rep_seq_y=[0 0.5*Tpwm 0]
  Sabc Pulse : Subsystem
  Scope : Scope  NumInputPorts=6
  Scope1 : Scope
  T1 T2 Caculate : Subsystem
  Tc Caculate : Subsystem
  Ts : Constant  Value=Tpwm
  "Udc " : Constant  Value=Vdc
  XYZ Caculate : Subsystem
  Pulse : Outport  VectorParamsAs1DForOutWhenUnconnected=off
  wires:
  beta/1 -> N Caculate/1(beta), XYZ Caculate/1(beta)
  alpha/1 -> N Caculate/2(alpha), XYZ Caculate/2(alpha)
  XYZ Caculate/1(X) -> T1 T2 Caculate/1(X)
  XYZ Caculate/2(Y) -> T1 T2 Caculate/2(Y)
  XYZ Caculate/3(Z) -> T1 T2 Caculate/3(Z)
  Ts/1 -> XYZ Caculate/3("Ts "), Tc Caculate/3(Ts), T1 T2 Caculate/5("Ts ")
  T1 T2 Caculate/1(T1) -> Tc Caculate/1(T1)
  T1 T2 Caculate/2(T2) -> Tc Caculate/2(T2)
  Tc Caculate/3(Tc3) -> Sabc Pulse/3(Tc3)
  Sabc Pulse/1("Pulse ") -> Demux/1, Pulse/1
  "Udc "/1 -> XYZ Caculate/4(Udc)
  Repeating Sequence/1 -> Sabc Pulse/4(Wave)
  Demux/1 -> Scope/1
  Demux/2 -> Scope/2
  Demux/3 -> Scope/3
  Demux/4 -> Scope/4
  Demux/5 -> Scope/5
  Demux/6 -> Scope/6
  N Caculate/1(N) -> Scope1/1, Tc Caculate/4(N), T1 T2 Caculate/4(N)
  Tc Caculate/2(Tc2) -> Sabc Pulse/2(Tc2)
  Tc Caculate/1(Tc1) -> Sabc Pulse/1(Tc1)

== system reduce_emf_before_speedloop/Subsystem/PI ==
  deta : Inport
  Add : Sum
  Discrete-Time Integrator : DiscreteIntegrator  SampleTime=-1  ICPrevOutput=DiscIntNeverNeededParam  ICPrevScaledInput=DiscIntNeverNeededParam
  ki : Gain  Gain=wn^2
  kp : Gain  Gain=2*wn
  we : Outport
  wires:
  ki/1 -> Discrete-Time Integrator/1
  deta/1 -> kp/1, ki/1
  Discrete-Time Integrator/1 -> Add/1
  kp/1 -> Add/2
  Add/1 -> we/1

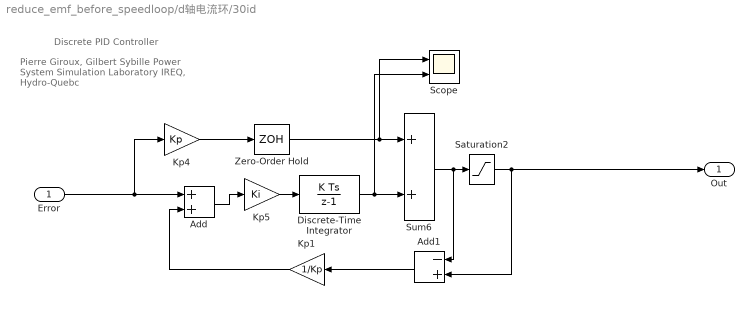
== system reduce_emf_before_speedloop/d轴电流环/30id ==
  note: Discrete PID Controller
  note: Pierre Giroux, Gilbert Sybille
      | Power System Simulation Laboratory
      | IREQ, Hydro-Quebc
  Error : Inport  SampleTime=Ts
  Add : Sum
  Add1 : Sum  Inputs=-+
  Discrete-Time Integrator : DiscreteIntegrator  InitialCondition=Init  SampleTime=Ts  LimitOutput=on  UpperSaturationLimit=UpperLimit  LowerSaturationLimit=LowerLimit  ICPrevOutput=DiscIntNeverNeededParam  ICPrevScaledInput=DiscIntNeverNeededParam
  Kp1 : Gain  Gain=1/Kp  SaturateOnIntegerOverflow=on  SampleTime=Ts  OutDataTypeStr=Inherit: Same as input  ParamDataTypeStr=Inherit: Same as input
  Kp4 : Gain  Gain=Kp  SaturateOnIntegerOverflow=on  SampleTime=Ts  OutDataTypeStr=Inherit: Same as input  ParamDataTypeStr=Inherit: Same as input
  Kp5 : Gain  Gain=Ki  SaturateOnIntegerOverflow=on  SampleTime=Ts  OutDataTypeStr=Inherit: Same as input  ParamDataTypeStr=Inherit: Same as input
  Saturation2 : Saturate  UpperLimit=UpperLimit  LowerLimit=LowerLimit  SampleTime=Ts
  Scope : Scope  NumInputPorts=2
  Sum6 : Sum  InputSameDT=on  SaturateOnIntegerOverflow=on  SampleTime=Ts  OutDataTypeStr=Inherit: Same as first input
  Zero-Order Hold : ZeroOrderHold  SampleTime=Ts
  Out : Outport  SampleTime=Ts  InitialOutput=0
  wires:
  Error/1 -> Kp4/1, Add/1
  Kp5/1 -> Discrete-Time Integrator/1
  Discrete-Time Integrator/1 -> Scope/2, Sum6/2
  Kp4/1 -> Zero-Order Hold/1
  Kp1/1 -> Add/2
  Add1/1 -> Kp1/1
  Sum6/1 -> Add1/1, Saturation2/1
  Add/1 -> Kp5/1
  Saturation2/1 -> Add1/2, Out/1
  Zero-Order Hold/1 -> Scope/1, Sum6/1

== system reduce_emf_before_speedloop/q轴电流环/30iq ==
  note: Discrete PID Controller
  note: Pierre Giroux, Gilbert Sybille
      | Power System Simulation Laboratory
      | IREQ, Hydro-Quebc
  Error : Inport  SampleTime=Ts
  Add : Sum
  Add1 : Sum  Inputs=-+
  Discrete-Time Integrator : DiscreteIntegrator  InitialCondition=Init  SampleTime=Ts  LimitOutput=on  UpperSaturationLimit=UpperLimit  LowerSaturationLimit=LowerLimit  ICPrevOutput=DiscIntNeverNeededParam  ICPrevScaledInput=DiscIntNeverNeededParam
  Kp1 : Gain  Gain=1/Kp  SaturateOnIntegerOverflow=on  SampleTime=Ts  OutDataTypeStr=Inherit: Same as input  ParamDataTypeStr=Inherit: Same as input
  Kp4 : Gain  Gain=Kp  SaturateOnIntegerOverflow=on  SampleTime=Ts  OutDataTypeStr=Inherit: Same as input  ParamDataTypeStr=Inherit: Same as input
  Kp5 : Gain  Gain=Ki  SaturateOnIntegerOverflow=on  SampleTime=Ts  OutDataTypeStr=Inherit: Same as input  ParamDataTypeStr=Inherit: Same as input
  Saturation2 : Saturate  UpperLimit=UpperLimit  LowerLimit=LowerLimit  SampleTime=Ts
  Scope : Scope  NumInputPorts=2
  Sum6 : Sum  InputSameDT=on  SaturateOnIntegerOverflow=on  SampleTime=Ts  OutDataTypeStr=Inherit: Same as first input
  Zero-Order Hold : ZeroOrderHold  SampleTime=Ts
  Out : Outport  SampleTime=Ts  InitialOutput=0
  wires:
  Zero-Order Hold/1 -> Scope/1, Sum6/1
  Discrete-Time Integrator/1 -> Scope/2, Sum6/2
  Kp4/1 -> Zero-Order Hold/1
  Kp5/1 -> Discrete-Time Integrator/1
  Sum6/1 -> Add1/1, Saturation2/1
  Error/1 -> Kp4/1, Add/1
  Saturation2/1 -> Add1/2, Out/1
  Add1/1 -> Kp1/1
  Add/1 -> Kp5/1
  Kp1/1 -> Add/2

== system reduce_emf_before_speedloop/转速环/30speed ==
  note: Discrete PID Controller
  note: Pierre Giroux, Gilbert Sybille
      | Power System Simulation Laboratory
      | IREQ, Hydro-Quebc
  Error : Inport  SampleTime=Ts
  Add : Sum
  Add1 : Sum  Inputs=-+
  Discrete-Time Integrator : DiscreteIntegrator  InitialCondition=Init  SampleTime=Ts  UpperSaturationLimit=UpperLimit  LowerSaturationLimit=LowerLimit  ICPrevOutput=DiscIntNeverNeededParam  ICPrevScaledInput=DiscIntNeverNeededParam
  Kp1 : Gain  Gain=1/Kp  SaturateOnIntegerOverflow=on  SampleTime=Ts  OutDataTypeStr=Inherit: Same as input  ParamDataTypeStr=Inherit: Same as input
  Kp4 : Gain  Gain=Kp  SaturateOnIntegerOverflow=on  SampleTime=Ts  OutDataTypeStr=Inherit: Same as input  ParamDataTypeStr=Inherit: Same as input
  Kp5 : Gain  Gain=Ki  SaturateOnIntegerOverflow=on  SampleTime=Ts  OutDataTypeStr=Inherit: Same as input  ParamDataTypeStr=Inherit: Same as input
  Saturation2 : Saturate  UpperLimit=UpperLimit  LowerLimit=LowerLimit  SampleTime=Ts
  Sum6 : Sum  InputSameDT=on  SaturateOnIntegerOverflow=on  SampleTime=Ts  OutDataTypeStr=Inherit: Same as first input
  Zero-Order Hold : ZeroOrderHold  SampleTime=Ts
  Out : Outport  SampleTime=Ts  InitialOutput=0
  wires:
  Kp1/1 -> Add/2
  Add1/1 -> Kp1/1
  Add/1 -> Kp5/1
  Zero-Order Hold/1 -> Sum6/1
  Discrete-Time Integrator/1 -> Sum6/2
  Kp4/1 -> Zero-Order Hold/1
  Kp5/1 -> Discrete-Time Integrator/1
  Error/1 -> Kp4/1, Add/1
  Sum6/1 -> Saturation2/1, Add1/1
  Saturation2/1 -> Out/1, Add1/2

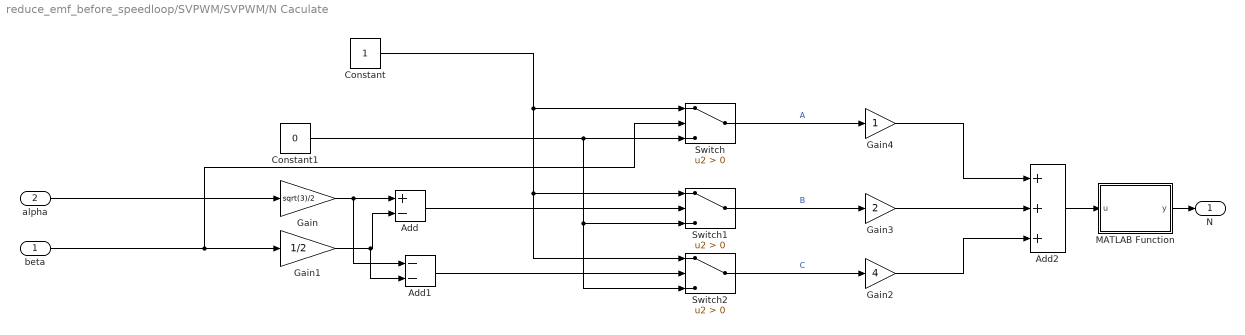
== system reduce_emf_before_speedloop/SVPWM/SVPWM/N Caculate ==
  beta : Inport
  alpha : Inport  Port=2
  Add : Sum  Inputs=+-
  Add1 : Sum  Inputs=--
  Add2 : Sum  Inputs=+++
  Constant : Constant
  Constant1 : Constant  Value=0
  Gain : Gain  Gain=sqrt(3)/2
  Gain1 : Gain  Gain=1/2
  Gain2 : Gain  Gain=4
  Gain3 : Gain  Gain=2
  Gain4 : Gain
  MATLAB Function : MATLAB Function  TreatAsAtomicUnit=on
  Switch : Switch  Criteria=u2 > Threshold  SaturateOnIntegerOverflow=off  InputSameDT=off
  Switch1 : Switch  Criteria=u2 > Threshold  SaturateOnIntegerOverflow=off  InputSameDT=off
  Switch2 : Switch  Criteria=u2 > Threshold  SaturateOnIntegerOverflow=off  InputSameDT=off
  N : Outport  VectorParamsAs1DForOutWhenUnconnected=off
  wires:
  Switch/1 -> Gain4/1  "A"
  Add/1 -> Switch1/2
  Gain/1 -> Add1/1, Add/1
  Gain3/1 -> Add2/2
  Gain2/1 -> Add2/3
  Constant/1 -> Switch/1, Switch2/1, Switch1/1
  Add1/1 -> Switch2/2
  Gain1/1 -> Add1/2, Add/2
  Add2/1 -> MATLAB Function/1(u)
  Constant1/1 -> Switch2/3, Switch1/3, Switch/3
  Gain4/1 -> Add2/1
  beta/1 -> Switch/2, Gain1/1
  Switch2/1 -> Gain2/1  "C"
  Switch1/1 -> Gain3/1  "B"
  alpha/1 -> Gain/1
  MATLAB Function/1(y) -> N/1

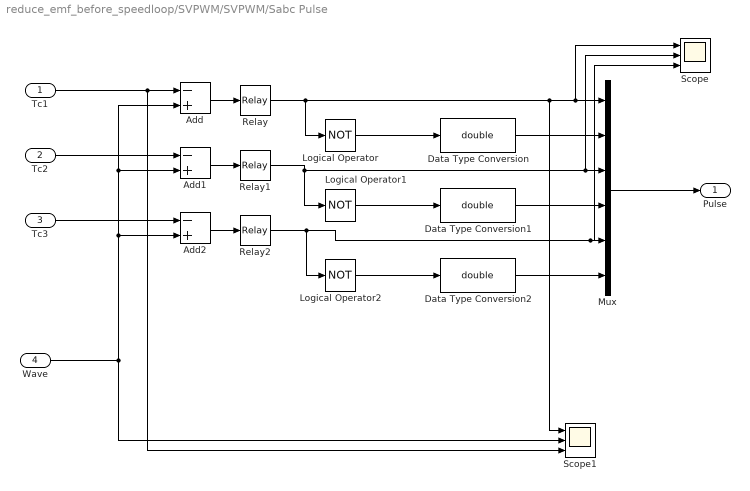
== system reduce_emf_before_speedloop/SVPWM/SVPWM/Sabc Pulse ==
  Tc1 : Inport
  Tc2 : Inport  Port=2
  Tc3 : Inport  Port=3
  Wave : Inport  Port=4
  Add : Sum  Inputs=-+
  Add1 : Sum  Inputs=-+
  Add2 : Sum  Inputs=-+
  Data Type Conversion : DataTypeConversion  OutDataTypeStr=double  SaturateOnIntegerOverflow=off  RndMeth=Floor
  Data Type Conversion1 : DataTypeConversion  OutDataTypeStr=double  SaturateOnIntegerOverflow=off  RndMeth=Floor
  Data Type Conversion2 : DataTypeConversion  OutDataTypeStr=double  SaturateOnIntegerOverflow=off  RndMeth=Floor
  Logical Operator : Logic  Operator=NOT  AllPortsSameDT=off  OutDataTypeStr=boolean
  Logical Operator1 : Logic  Operator=NOT  AllPortsSameDT=off  OutDataTypeStr=boolean
  Logical Operator2 : Logic  Operator=NOT  AllPortsSameDT=off  OutDataTypeStr=boolean
  Mux : Mux  Inputs=6
  Relay : Relay
  Relay1 : Relay
  Relay2 : Relay
  Scope : Scope  NumInputPorts=3
  Scope1 : Scope  NumInputPorts=3
  "Pulse " : Outport  VectorParamsAs1DForOutWhenUnconnected=off
  wires:
  Add/1 -> Relay/1
  Add1/1 -> Relay1/1
  Wave/1 -> Add2/2, Add1/2, Add/2, Scope1/2
  Tc2/1 -> Add1/1
  Tc1/1 -> Scope1/3, Add/1
  Tc3/1 -> Add2/1
  Logical Operator/1 -> Data Type Conversion/1
  Logical Operator1/1 -> Data Type Conversion1/1
  Add2/1 -> Relay2/1
  Logical Operator2/1 -> Data Type Conversion2/1
  Mux/1 -> "Pulse "/1
  Relay/1 -> Scope1/1, Scope/1, Mux/1, Logical Operator/1
  Relay1/1 -> Scope/2, Mux/3, Logical Operator1/1
  Relay2/1 -> Logical Operator2/1, Scope/3, Mux/5
  Data Type Conversion/1 -> Mux/2
  Data Type Conversion1/1 -> Mux/4
  Data Type Conversion2/1 -> Mux/6

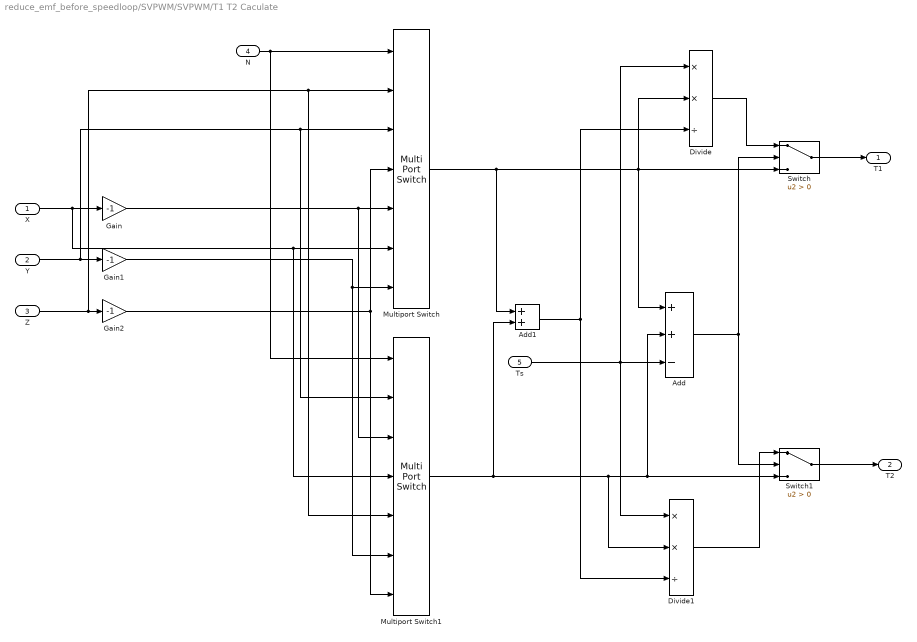
== system reduce_emf_before_speedloop/SVPWM/SVPWM/T1 T2 Caculate ==
  X : Inport
  Y : Inport  Port=2
  Z : Inport  Port=3
  N : Inport  Port=4
  "Ts " : Inport  Port=5
  Add : Sum  Inputs=++-
  Add1 : Sum
  Divide : Product  Inputs=**/
  Divide1 : Product  Inputs=**/
  Gain : Gain  Gain=-1
  Gain1 : Gain  Gain=-1
  Gain2 : Gain  Gain=-1
  Multiport Switch : MultiPortSwitch  Inputs=6  SaturateOnIntegerOverflow=off  InputSameDT=off
  Multiport Switch1 : MultiPortSwitch  Inputs=6  SaturateOnIntegerOverflow=off  InputSameDT=off
  Switch : Switch  Criteria=u2 > Threshold  SaturateOnIntegerOverflow=off  InputSameDT=off
  Switch1 : Switch  Criteria=u2 > Threshold  SaturateOnIntegerOverflow=off  InputSameDT=off
  T1 : Outport  VectorParamsAs1DForOutWhenUnconnected=off
  T2 : Outport  Port=2  VectorParamsAs1DForOutWhenUnconnected=off
  wires:
  Y/1 -> Multiport Switch1/2, Multiport Switch/3, Gain1/1
  X/1 -> Multiport Switch1/4, Multiport Switch/6, Gain/1
  N/1 -> Multiport Switch/1, Multiport Switch1/1
  Z/1 -> Multiport Switch1/5, Multiport Switch/2, Gain2/1
  Gain2/1 -> Multiport Switch1/7, Multiport Switch/4
  Gain/1 -> Multiport Switch1/3, Multiport Switch/5
  Gain1/1 -> Multiport Switch1/6, Multiport Switch/7
  Multiport Switch/1 -> Add1/1, Divide/2, Add/1, Switch/3
  Multiport Switch1/1 -> Add1/2, Divide1/2, Add/2, Switch1/3
  "Ts "/1 -> Divide1/1, Divide/1, Add/3
  Add/1 -> Switch1/2, Switch/2
  Divide/1 -> Switch/1
  Add1/1 -> Divide/3, Divide1/3
  Switch/1 -> T1/1
  Switch1/1 -> T2/1
  Divide1/1 -> Switch1/1

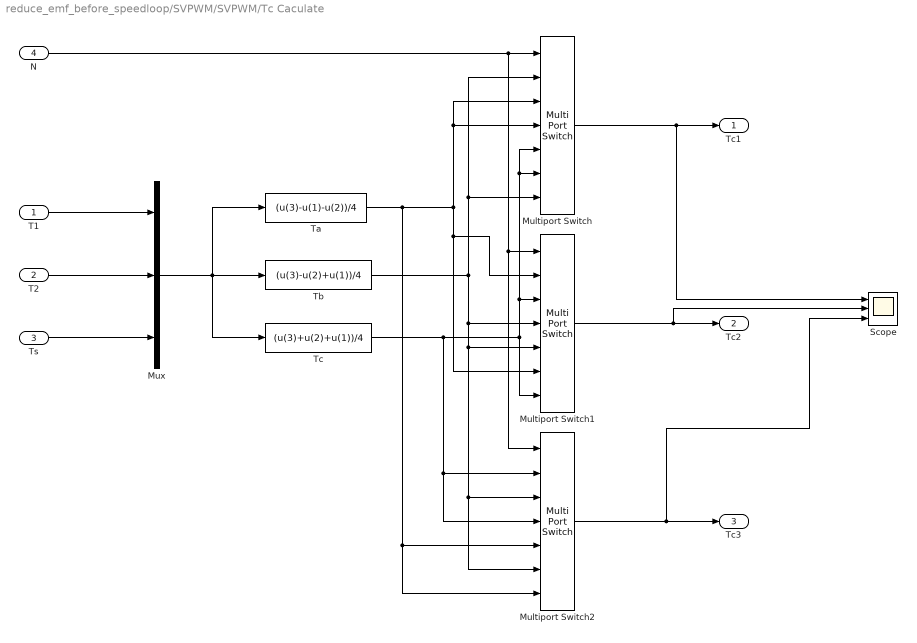
== system reduce_emf_before_speedloop/SVPWM/SVPWM/Tc Caculate ==
  T1 : Inport
  T2 : Inport  Port=2
  Ts : Inport  Port=3
  N : Inport  Port=4
  Multiport Switch : MultiPortSwitch  Inputs=6  SaturateOnIntegerOverflow=off  InputSameDT=off
  Multiport Switch1 : MultiPortSwitch  Inputs=6  SaturateOnIntegerOverflow=off  InputSameDT=off
  Multiport Switch2 : MultiPortSwitch  Inputs=6  SaturateOnIntegerOverflow=off  InputSameDT=off
  Mux : Mux  Inputs=3
  Scope : Scope  NumInputPorts=3
  Ta : Fcn  Expr=(u(3)-u(1)-u(2))/4
  Tb : Fcn  Expr=(u(3)-u(2)+u(1))/4
  Tc : Fcn  Expr=(u(3)+u(2)+u(1))/4
  Tc1 : Outport  VectorParamsAs1DForOutWhenUnconnected=off
  Tc2 : Outport  Port=2  VectorParamsAs1DForOutWhenUnconnected=off
  Tc3 : Outport  Port=3  VectorParamsAs1DForOutWhenUnconnected=off
  wires:
  T2/1 -> Mux/2
  T1/1 -> Mux/1
  Ts/1 -> Mux/3
  Mux/1 -> Tc/1, Ta/1, Tb/1
  N/1 -> Multiport Switch2/1, Multiport Switch1/1, Multiport Switch/1
  Ta/1 -> Multiport Switch2/7, Multiport Switch2/5, Multiport Switch/3, Multiport Switch/4, Multiport Switch1/6, Multiport Switch1/2
  Tb/1 -> Multiport Switch/7, Multiport Switch/2, Multiport Switch1/4, Multiport Switch2/6, Multiport Switch2/3, Multiport Switch1/5
  Tc/1 -> Multiport Switch2/4, Multiport Switch2/2, Multiport Switch1/7, Multiport Switch1/3, Multiport Switch/6, Multiport Switch/5
  Multiport Switch/1 -> Scope/1, Tc1/1
  Multiport Switch1/1 -> Scope/2, Tc2/1
  Multiport Switch2/1 -> Scope/3, Tc3/1

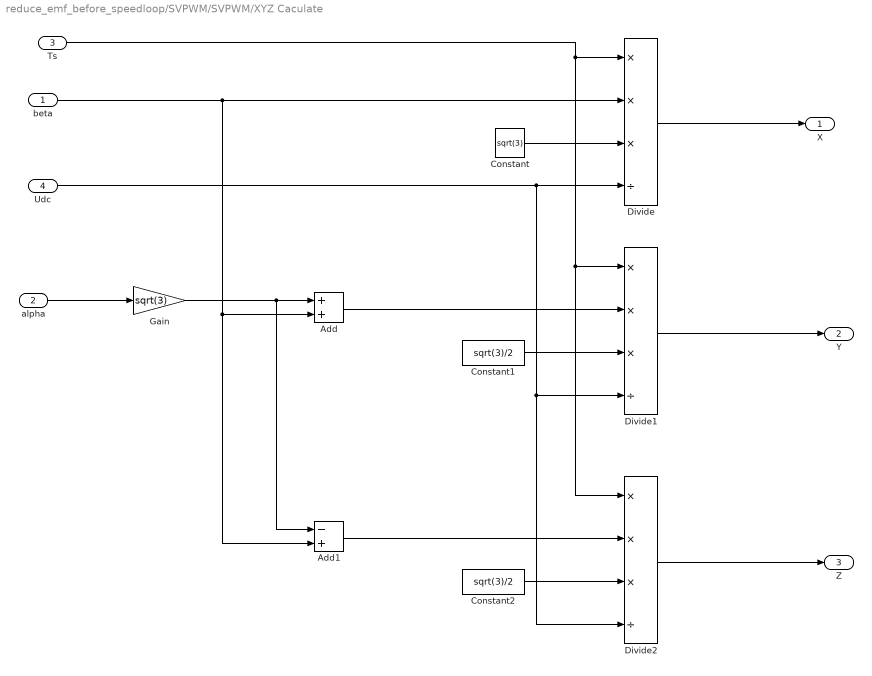
== system reduce_emf_before_speedloop/SVPWM/SVPWM/XYZ Caculate ==
  beta : Inport
  alpha : Inport  Port=2
  "Ts " : Inport  Port=3
  Udc : Inport  Port=4
  Add : Sum
  Add1 : Sum  Inputs=-+
  Constant : Constant  Value=sqrt(3)
  Constant1 : Constant  Value=sqrt(3)/2
  Constant2 : Constant  Value=sqrt(3)/2
  Divide : Product  Inputs=***/
  Divide1 : Product  Inputs=***/
  Divide2 : Product  Inputs=***/
  Gain : Gain  Gain=sqrt(3)
  X : Outport  VectorParamsAs1DForOutWhenUnconnected=off
  Y : Outport  Port=2  VectorParamsAs1DForOutWhenUnconnected=off
  Z : Outport  Port=3  VectorParamsAs1DForOutWhenUnconnected=off
  wires:
  "Ts "/1 -> Divide2/1, Divide1/1, Divide/1
  Udc/1 -> Divide1/4, Divide2/4, Divide/4
  Constant/1 -> Divide/3
  beta/1 -> Add1/2, Add/2, Divide/2
  Constant2/1 -> Divide2/3
  Constant1/1 -> Divide1/3
  Add/1 -> Divide1/2
  Add1/1 -> Divide2/2
  Gain/1 -> Add1/1, Add/1
  alpha/1 -> Gain/1
  Divide1/1 -> Y/1
  Divide/1 -> X/1
  Divide2/1 -> Z/1

== matlab function reduce_emf_before_speedloop/参数辨识与采集/参数辨识 ==
  settings: updateMethod=DISCRETE  sampleTime=1e-4
  data: ud input; y output; uq input; id input; err1 output; err2 output; iq input; we input; Vstate input
function [y,err1,err2] = fcn(ud,uq,id,iq,we,Vstate)
%#codegen
% 论文式12.25～12.28：两组位置误差与逐样本递推最小二乘辨识。
% 输入为五路同周期、同系数的50 Hz低通信号，采样周期均为100微秒。
% 在辨识支路内对五路信号使用相同的一电周期滑动平均，抑制周期纹波。
% 调试版：窗口填满即保存；稳态、工作点、角度及条件数仅提示，不阻断。
% y(5)、y(7)表示数值计算完成，不代表已经通过精度或物理合理性验收。
% y(17)保留首个诊断提示；18～27列为电压诊断，未计算参数为NaN。
persistent buf count oldState ready result aerr berr finished
persistent angleK angDone sumDiff m theta P iteration checked window cursor filled
persistent cycleBuf cycleSum cycleHead cycleCount cycleN rawWindow
if isempty(count)
    buf=zeros(2000,5,6); count=0; oldState=-1; ready=false(6,1);
    result=zeros(27,1); result([3 4 6])=NaN;
    aerr=zeros(400,1); berr=zeros(400,1);
    finished=false; angleK=0; angDone=false; sumDiff=zeros(2,2);
    m=zeros(6,5); theta=zeros(2,1); P=10*eye(2);
    iteration=0; checked=false; window=zeros(2000,5); cursor=0; filled=0;
    cycleBuf=zeros(1257,5); cycleSum=zeros(1,5);
    cycleHead=0; cycleCount=0; cycleN=1; rawWindow=zeros(2000,2);
end
u=[ud uq id iq we];
if ~all(isfinite(u)) || ~isfinite(Vstate)
    ready(:)=false; result(:)=0; result([3 4 6])=NaN;
    result(8)=-1; result(17)=-1;
    if Vstate>=2 && Vstate<=8, result(16)=-Vstate; end
    finished=true; y=result; err1=aerr; err2=berr; return;
end
if Vstate~=oldState
    count=0; oldState=Vstate; cursor=0; filled=0; result(16)=0;
    cycleBuf(:)=0; cycleSum(:)=0; cycleHead=0; cycleCount=0; cycleN=1;
    if Vstate==0 || Vstate==2
        ready(:)=false; result(:)=0; result([3 4 6])=NaN;
        aerr(:)=0; berr(:)=0;
        finished=false; angleK=0; angDone=false; sumDiff(:)=0;
        theta(:)=0; P=10*eye(2); iteration=0; checked=false;
    end
end
slot=0;
if Vstate==2, slot=1;
elseif Vstate==3, slot=2;
elseif Vstate==4, slot=3;
elseif Vstate==6, slot=4;
elseif Vstate==7, slot=5;
elseif Vstate==8, slot=6;
end
if slot>0 && ~ready(slot) && ~finished
    result(8)=1; count=count+1; result(15)=count;
    result(27)=Vstate;
    % 阶段开始0.1秒后，用滤波后的电角速度确定一电周期长度并锁存。
    % N约等于2π/(|we|*Ts)。只对辨识数据处理，不改变控制环及任务周期。
    % 每次切换阶段均清空平均器，防止混入上一个注入状态的数据。
    if count==1000
        cycleN=min(1257,max(50,round(2*pi/(max(abs(we),50)*1e-4))));
        cycleBuf(:)=0; cycleSum(:)=0; cycleHead=0; cycleCount=0;
    end
    smooth=u;
    if count>=1000
        cycleHead=mod(cycleHead,cycleN)+1;
        cycleSum=cycleSum+u-cycleBuf(cycleHead,:);
        cycleBuf(cycleHead,:)=u; cycleCount=min(cycleN,cycleCount+1);
        smooth=cycleSum/cycleCount;
    end
    result(26)=cycleN;
    % 至少等待0.2秒，并确保周期平均器已填满，再保存最新0.2秒窗口。
    % 调试版不再等待窗口通过验收；窗口填满后即存储，PLL按固定时长推进。
    if count>max(2000,999+cycleN)
        cursor=mod(cursor,2000)+1; window(cursor,:)=smooth;
        rawWindow(cursor,:)=u(1:2);
        filled=min(2000,filled+1);
    end
    if filled==2000 && mod(count,200)==0
        W=zeros(2000,5);
        for n=1:2000, W(n,:)=window(mod(cursor+n-1,2000)+1,:); end
        [meanW,reason,drift,diagV]=check_window(W);
        result(10)=drift;
        rawMean=sum(rawWindow,1)/2000;
        for j=1:2
            result(17+j)=sqrt(sum((rawWindow(:,j)-rawMean(j)).^2)/2000);
        end
        result(20:25)=diagV;
        if slot~=1 && slot~=4
            base=1+3*(slot>3);
            mismatch=norm(meanW(3:4)-m(base,3:4));
            result(11)=max(result(11),mismatch);
            if mismatch>max(0.02,0.005*norm(m(base,3:4))) || ...
                    abs(meanW(5)-m(base,5))>max(1,0.005*abs(m(base,5)))
                if reason==0, reason=-6; end
            end
        end
        % 正负窗口差异仅记录提示，按用户要求先输出实际数据的辨识曲线。
        if slot==3 || slot==6
            plus=slot-1;
            if norm(meanW(3:4)-m(plus,3:4))>max(0.003,0.0005*norm(m(plus,3:4))) || ...
                    abs(meanW(5)-m(plus,5))>max(0.02,0.0001*abs(m(plus,5)))
                if reason==0, reason=-12; end
            end
        end
        if result(17)==0 && reason~=0, result(17)=reason; end
        buf(:,:,slot)=W; m(slot,:)=meanW; ready(slot)=true;
        result(16)=Vstate;
    end
end
if Vstate==10 && ~finished
    result(8)=-10; result(17)=-10; finished=true;
end
if Vstate==9 && ~finished
    if ~all(ready)
        result(8)=-2; result(17)=-2; finished=true;
    elseif ~checked
        checked=true; result(8)=2;
    elseif ~angDone
        % 位置误差更新400次，每次消耗五个尚未处理的存储样本。
        angleK=angleK+1;
        for g=1:2
            pos=2+3*(g-1); neg=pos+1;
            for n=(angleK-1)*5+1:angleK*5
                sumDiff(g,1)=sumDiff(g,1)+buf(n,1,pos)-buf(n,1,neg);
                sumDiff(g,2)=sumDiff(g,2)+buf(n,2,pos)-buf(n,2,neg);
            end
            d=atan2(sumDiff(g,2),sumDiff(g,1));
            if d>pi/2, d=d-pi; elseif d< -pi/2, d=d+pi; end
            result(g)=d;
            if g==1, aerr(angleK)=d; else, berr(angleK)=d; end
        end
        if angleK==400
            angDone=true;
            for g=1:2
                if norm(sumDiff(g,:))/2000<0.2 || abs(result(g))>0.6
                    if result(17)==0, result(17)=-7; end
                end
            end
            % 条件数仅用于诊断，不在此处预先求解参数，也不阻止递推。
            H=zeros(2,2);
            for g=1:2
                b=1+3*(g-1); di=m(b,3); qi=m(b,4); w=m(b,5);
                row=[0.01*w*(di^2+qi^2), ...
                    0.2*w*(di*cos(result(g))+qi*sin(result(g)))];
                H(g,:)=row/max(norm(row),1e-12);
            end
            detH=H(1,1)*H(2,2)-H(1,2)*H(2,1);
            tau=sum(sum(H.^2));
            condH=(tau+sqrt(max(0,tau*tau-4*detH*detH)))/(2*max(abs(detH),1e-12));
            result(9)=condH;
            if condH>100 || abs(detH)<1e-6
                if result(17)==0, result(17)=-8; end
            end
        end
    else
        % 按A1、B1、A2、B2……A2000、B2000顺序读取两组基准数据。
        % 每次调用只使用一个观测量，执行一次实际递推，不反复重放同一批数据。
        % 正负注入数据用于估计位置误差，基准数据用于L和磁链辨识。
        iteration=iteration+1;
        g=1+mod(iteration-1,2); n=floor((iteration-1)/2)+1;
        b=1+3*(g-1); di=buf(n,3,b); qi=buf(n,4,b); w=buf(n,5,b);
        raw=[0.01*w*(di^2+qi^2); ...
            0.2*w*(di*cos(result(g))+qi*sin(result(g)))];
        scale=max(norm(raw),1e-12); phi=raw/scale;
        voltage=(buf(n,2,b)*di-buf(n,1,b)*qi)/scale;
        gain=P*phi/(1+phi'*P*phi);
        innovation=voltage-phi'*theta;
        theta=theta+gain*innovation;
        % 用Joseph形式更新协方差，测量方差及遗忘因子均为1。
        % 滑动平均后的相邻样本存在相关性，协方差不解释为统计置信区间。
        A=eye(2)-gain*phi'; P=A*P*A'+gain*gain'; P=0.5*(P+P');
        result(3)=0.01*theta(1); result(4)=0.2*theta(2);
        result(8)=3; result(12)=iteration; result(13)=innovation;
        % 每次L和磁链递推后同步计算Rs，不因物理范围或相对门限隐藏结果。
        D=zeros(2,1); z=zeros(2,1);
        for h=1:2
            bb=1+3*(h-1); dd=m(bb,3); qq=m(bb,4); ww=m(bb,5);
            D(h)=(4/pi)*qq/max(hypot(dd,qq),1e-8);
            z(h)=m(bb,2)-ww*result(3)*dd-ww*result(4)*cos(result(h));
        end
        den=D(2)*m(1,4)-D(1)*m(4,4);
        rsScale=abs(D(2)*m(1,4))+abs(D(1)*m(4,4));
        result(14)=abs(den)/max(rsScale,1e-12);
        % 仅保留浮点除零保护；不可求时保留NaN，不用额定值代替结果。
        canDivide=abs(den)>64*eps(max(rsScale,1));
        if canDivide
            result(6)=(D(2)*z(1)-D(1)*z(2))/den;
        else
            result(6)=NaN;
        end
        if iteration==4000
            finished=true;
            result(5)=double(all(isfinite(theta)));
            result(7)=double(isfinite(result(6)));
            result(8)=30;
            if result(7)==0 && result(17)==0, result(17)=-11; end
        end
    end
end
y=result; err1=aerr; err2=berr;
end

function [meanW,reason,maxDrift,diagV] = check_window(W)
% 仅计算诊断提示，不拒绝窗口、不超时中止、不抑制参数输出。
% 原始纹波先经相同的电周期平均；慢漂移不会被此单位直流增益滤波消除。
% 诊断六列依次为：ud/uq剩余标准差、ud/uq漂移门限比、ud/uq纹波门限比。
meanW=sum(W,1)/2000; reason=0; maxDrift=0;
diagV=zeros(6,1);
for j=1:5
    sd=sqrt(sum((W(:,j)-meanW(j)).^2)/2000);
    drift=abs(sum(W(1:1000,j))/1000-sum(W(1001:2000,j))/1000);
    if j<=2
        st=max(0.10,0.005*abs(meanW(j)));
        dt=max(0.05,0.002*norm(meanW(1:2)));
        maxDrift=max(maxDrift,drift); code=-13;
        diagV(j)=sd; diagV(2+j)=drift/dt; diagV(4+j)=sd/st;
        % -3只表示均值仍在慢漂移；-13表示周期平均后仍有过大纹波。
        if drift>dt && (reason==0 || reason==-13), reason=-3; end
    elseif j<=4
        st=max(0.01,0.005*norm(meanW(3:4)));
        dt=max(0.015,0.005*norm(meanW(3:4))); code=-4;
    else
        st=max(0.3,0.002*abs(meanW(j)));
        dt=max(0.5,0.003*abs(meanW(j))); code=-5;
    end
    if (sd>st || drift>dt) && reason==0, reason=code; end
end
if abs(meanW(5))<50 && reason==0, reason=-5; end
end

== matlab function reduce_emf_before_speedloop/SVPWM/SVPWM/N Caculate/MATLAB Function ==
  data: u input; y output
function y = fcn(u)
if u==0
    y=1;
else
    y = u;
end

== matlab function reduce_emf_before_speedloop/MATLAB Function2 ==
  data: n input; n_filt output
function n_filt = fcn(n)
%#codegen
% 五路共用相同的50 Hz低通；周期平均在参数辨识函数内部执行。
n_filt=n;
end

== matlab function reduce_emf_before_speedloop/MATLAB Function1 ==
  data: n input; n_filt output
function n_filt = fcn(n)
%#codegen
% 文档图12.2的PLL速度反馈接口；输入来自原有一拍延迟的PLL速度。
% 本版旁路原100Hz低通，确保角度推进与解耦使用同一拍速度。
n_filt = n;
end

== matlab function reduce_emf_before_speedloop/Subsystem/MATLAB Function1 ==
  data: u input; y output; deta input
function y = fcn(u,deta)
a=1e-6;
if u<a
    y=0;
else
    y=deta;
end
